simulink model "chbtask"  (R2024b)
settings: Solver=FixedStepDiscrete  StartTime=0.0  StopTime=0.2  FixedStep=5e-5  RelTol=1e-3
values from neighbouring files (symbols this model uses):
  CHB_MODE : value not decoded    [CHB_Data.sldd]
  INV120_CUURENTLOOP_KP = 2.0    [CHB_Data.sldd]
  INV120_CUURENTLOOP_KR = 5.0    [CHB_Data.sldd]
  INV120_VOLTAGELOOP_KI = 0.005    [CHB_Data.sldd]
  INV120_VOLTAGELOOP_KP = 0.5    [CHB_Data.sldd]
  INV240_VOLTAGELOOP_KI = 0.005    [CHB_Data.sldd]
  INV240_VOLTAGELOOP_KP = 0.5    [CHB_Data.sldd]
  PFC120_CUURENTLOOP_KP = 30.0    [CHB_Data.sldd]
  PFC120_CUURENTLOOP_KR = 8.0    [CHB_Data.sldd]
  PFC120_POWERLOOP_KI = 0.0001    [CHB_Data.sldd]
  PFC120_POWERLOOP_KP = 0.005    [CHB_Data.sldd]
  PFC240_CUURENTLOOP_KP = 5.0    [CHB_Data.sldd]
  PFC240_CUURENTLOOP_KR = 10.0    [CHB_Data.sldd]
  PFC240_POWERLOOP_KI = 0.0001    [CHB_Data.sldd]
  PFC240_POWERLOOP_KP = 0.005    [CHB_Data.sldd]
undefined symbols (not defined in the file or in its folder): Ii_rms, Io_rms, Io_rms_a, Io_rms_b, Vi_freq, Vi_rms, Vo_freq, Vo_freq_a, Vo_freq_b, Vo_rms, Vo_rms_a, Vo_rms_b
(part 3 of 3)

== stateflow chart chbtask/Algorithm_Ctrl/MainCtrl/inv120_func/inv120_en/Chart7 ==
  (default) -> (junction 3) : {
      | pi_out_value = single(1)*Pi_inv_out;
      | cnt = mod(cnt + 1, 200);
      | %PWM1 = sin_tab(mod(cnt + 0, 400) + 1);
      | out = pi_out_value*sin_wave(mod(cnt + 0, 200) + 1);
      | }
  data: sin_wave local single =[
0.000000000, 0.031410759, 0.062790520, 0.094108313, 0.125333234, 0.156434465, 0.187381315, 0.218143241, 0.248689887, 0.278991106, 0.309016994, 0.338737920, 0.368124553, 0.397147891, 0.425779292, 0.453990500, 0.481753674, 0.509041416, 0.535826795, 0.562083325, 0.587785252, 0.612907054, 0.637423990, 0.661311865, 0.684547106, 0.707106781, 0.728968627, 0.750111065, 0.770513243, 0.790155012, 0.809016994, 0.827080574, 0.844327926, 0.860742028, 0.876306680, 0.891006524, 0.904827052, 0.917754626, 0.929776486, 0.940880769, 0.951056516, 0.960293686, 0.968583162, 0.975916762, 0.982287251, 0.987688341, 0.992114701, 0.995561965, 0.998026728, 0.999506560, 1.000000000, 0.999506560, 0.998026728, 0.995561965, 0.992114701, 0.987688341, 0.982287251, 0.975916762, 0.968583162, 0.960293686, 0.951056516, 0.940880769, 0.929776486, 0.917754626, 0.904827052, 0.891006524, 0.876306680, 0.860742028, 0.844327926, 0.827080574, 0.809016994, 0.790155012, 0.770513243, 0.750111065, 0.728968627, 0.707106781, 0.684547106, 0.661311865, 0.637423990, 0.612907054, 0.587785252, 0.562083325, 0.535826795, 0.509041416, 0.481753674, 0.453990500, 0.425779292, 0.397147891, 0.368124553, 0.338737920, 0.309016994, 0.278991106, 0.248689887, 0.218143241, 0.187381315, 0.156434465, 0.125333234, 0.094108313, 0.062790520, 0.031410759, 0.000000000, -0.031410759, -0.062790520, -0.094108313, -0.125333234, -0.156434465, -0.187381315, -0.218143241, -0.248689887, -0.278991106, -0.309016994, -0.338737920, -0.368124553, -0.397147891, -0.425779292, -0.453990500, -0.481753674, -0.509041416, -0.535826795, -0.562083325, -0.587785252, -0.612907054, -0.637423990, -0.661311865, -0.684547106, -0.707106781, -0.728968627, -0.750111065, -0.770513243, -0.790155012, -0.809016994, -0.827080574, -0.844327926, -0.860742028, -0.876306680, -0.891006524, -0.904827052, -0.917754626, -0.929776486, -0.940880769, -0.951056516, -0.960293686, -0.968583162, -0.975916762, -0.982287251, -0.987688341, -0.992114701, -0.995561965, -0.998026728, -0.999506560, -1.000000000, -0.999506560, -0.998026728, -0.995561965, -0.992114701, -0.987688341, -0.982287251, -0.975916762, -0.968583162, -0.960293686, -0.951056516, -0.940880769, -0.929776486, -0.917754626, -0.904827052, -0.891006524, -0.876306680, -0.860742028, -0.844327926, -0.827080574, -0.809016994, -0.790155012, -0.770513243, -0.750111065, -0.728968627, -0.707106781, -0.684547106, -0.661311865, -0.637423990, -0.612907054, -0.587785252, -0.562083325, -0.535826795, -0.509041416, -0.481753674, -0.453990500, -0.425779292, -0.397147891, -0.368124553, -0.338737920, -0.309016994, -0.278991106, -0.248689887, -0.218143241, -0.187381315, -0.156434465, -0.125333234, -0.094108313, -0.062790520, -0.031410759
]; Pi_inv_out input single; cnt local single =0; out output single =0; pi_out_value local single =0

== stateflow chart chbtask/Task_Scheduler/Chart1 ==
  settings: executeAtInitialization=1
  (default) -> (junction 6)
  (junction 6) -> (junction 8) [order 1] : [cnt==0]
  (junction 6) -> (junction 11) [order 2] : {
      | out=0;
      | cnt=0;
      | }
  (junction 8) -> (junction 13) : {
      | out=1;
      | cnt=1;
      | }
  data: out output uint8 =0; cnt local uint8 =0
  events: event input FUNCTION_CALL_EVENT

== matlab function chbtask/Func/Rms/RMS ==
  data: Fs input single size=1; X_rms output single size=1; X_data input single size=1; limit_cnt input single size=[1 2]; pre_data input single size=[1 5]; X_freq output single size=1; out_data output single size=[1 5]
function [X_rms, X_freq, out_data] = RMS(Fs, X_data, limit_cnt, pre_data)
%%#codegen
sum_val = pre_data(1) + X_data * X_data; %均方根求和SUM
cnt = pre_data(2) + single(1); %cnt计数
prev = X_data;
out_data = [sum_val, cnt, prev, pre_data(4), pre_data(5)];

if (X_data > single(0)) && (pre_data(3) <= single(0)) && (cnt >= limit_cnt(1)) %过零点且采样点>最小限制
    temp = single(1) / cnt;
    X_freq = temp * Fs;
    X_rms = single(sqrt(double(temp * sum_val)));
    out_data(1) = single(0);
    out_data(2) = single(0);
    out_data(4) = X_rms;
    out_data(5) = X_freq;
elseif cnt > limit_cnt(2) %采样点>最大限制
    X_freq = single(0);
    X_rms = single(0);
    out_data(1) = single(0);
    out_data(2) = single(0);
    out_data(4) = single(0);
    out_data(5) = single(0);
else
    X_rms = pre_data(4);
    X_freq = pre_data(5);
end
end

== stateflow chart chbtask/Task_Scheduler/Chart ==
  state freq_divie
    %将系统频率分为20k、10k、5k、1k四个档次
    %%输出类型为事件触发
    cnt=cnt+1;
    %10k
    if (mod(cnt, 2)==0)
    freq_10k_flg1;
    elseif (mod(cnt, 2)==1)
    freq_10k_flg2;
    end
    %%5k
    if (mod(cnt, 4)==0)
    freq_05k_flg1;
    elseif(mod(cnt, 4)==1)
    freq_05k_flg2;
    elseif(mod(cnt, 4)==2)
    freq_5k_flg3;
    elseif(mod(cnt, 4)==3)
    freq_5k_flg4;
    elseif(mod(cnt, 4)==4)
    freq_5k_flg5;
    end
    %%1k
    if (mod(cnt, 20)==1)
    freq_01k_flg1;
    elseif(mod(cnt, 20)==2)
    freq_01k_flg2;
    elseif(mod(cnt, 20)==2)
    freq_01k_flg3;
    elseif(mod(cnt, 20)==2)
    freq_01k_flg4;
    elseif(mod(cnt, 20)==2)
    freq_01k_flg5;
    elseif(mod(cnt, 20)==0)
    cnt = 0;
    end
    freq_20k_flg;
  (default) -> freq_divie
  data: cnt local uint16 =0
  events: freq_01k_flg1 output FUNCTION_CALL_EVENT; freq_01k_flg2 output FUNCTION_CALL_EVENT; freq_01k_flg3 output FUNCTION_CALL_EVENT; freq_01k_flg4 output FUNCTION_CALL_EVENT; freq_01k_flg5 output FUNCTION_CALL_EVENT; freq_05k_flg1 output FUNCTION_CALL_EVENT; freq_05k_flg2 output FUNCTION_CALL_EVENT; freq_5k_flg3 output FUNCTION_CALL_EVENT; freq_5k_flg4 output FUNCTION_CALL_EVENT; freq_5k_flg5 output FUNCTION_CALL_EVENT; freq_10k_flg1 output FUNCTION_CALL_EVENT; freq_10k_flg2 output FUNCTION_CALL_EVENT; freq_20k_flg output FUNCTION_CALL_EVENT

== stateflow chart chbtask/SPWM_Table/SPWM_Chart ==
  state SPWM_gen
    entry:
    cnt = 0;
    during:
    cnt = mod(cnt + 1, 400);
    PWM1 = sin_tab(mod(cnt + 0, 400) + 1);
    PWM2 = 0.5 + 0.5*sin_tab(mod(cnt + 100, 400) + 1);
    PWM3 = 0.5 + 0.5*sin_tab(mod(cnt + 200, 400) + 1);
    PWM4 = 0.5 + 0.5*sin_tab(mod(cnt + 300, 400) + 1);
  data: PWM1 output single =0.5; PWM2 output single =0.99; PWM3 output single =0.5; PWM4 output single =0.01; cnt local int32; sin_tab local single =[0 0.0153931709655843 0.0307825438965657 0.0461643216954498 0.0615347091387271 0.076889913813288 0.092226147052144 0.107539624869224 0.122826568893018 0.138083207298831 0.153305775739426 0.168490518273821 0.18363368829401 0.198731549449382 0.213780376568612 0.228776456578787 0.243716089421558 0.258595588966065 0.273411283918445 0.288159518727658 0.302836654487448 0.317439069834186 0.331963161840386 0.346405346903672 0.360762061630984 0.375029763717788 0.389204932822085 0.403284071433007 0.417263705733771 0.431140386458797 0.444910689744756 0.458571217975362 0.472118600619681 0.485549495063759 0.498860587435364 0.51204859342163 0.525110259079417 0.538042361638169 0.550841710295088 0.563505147002413 0.576029547246624 0.588411820819366 0.600648912579917 0.612737803208991 0.624675509953716 0.63645908736358 0.648085628017179 0.659552263239578 0.670856163810115 0.681994540660468 0.692964645562816 0.703763771807925 0.714389254872983 0.724838473079037 0.73510884823785 0.74519784628803 0.755102977920273 0.764821799191563 0.774351912128177 0.783690965317349 0.792836654487448 0.801786723076523 0.810538962789071 0.819091214140905 0.827441366991975 0.83558736106701 0.843527186463865 0.851258884149428 0.858780546442986 0.86609031748692 0.8731863937046 0.880067024245403 0.886730511416699 0.893175211102736 0.899399533170302 0.905401941861061 0.911180956170486 0.91673515021327 0.922063153575141 0.927163651650994 0.93203538596925 0.936677154502364 0.941087811963404 0.945266270088642 0.949211497906058 0.952922521989723 0.956398426699972 0.95963835440933 0.962641505714115 0.965407139631678 0.967934573783235 0.970223184562226 0.972272407288188 0.974081736346076 0.975650725311018 0.976978987058465 0.978066193859706 0.978912077462731 0.979516429158417 0.979879099832027 0.98 0.979879099832027 0.979516429158417 0.978912077462731 0.978066193859706 0.976978987058465 0.975650725311018 0.974081736346076 0.972272407288188 0.970223184562226 0.967934573783235 0.965407139631678 0.962641505714115 0.95963835440933 0.956398426699972 0.952922521989723 0.949211497906058 0.945266270088642 0.941087811963404 0.936677154502364 0.932035385969251 0.927163651650994 0.922063153575141 0.91673515021327 0.911180956170486 0.905401941861061 0.899399533170302 0.893175211102736 0.886730511416699 0.880067024245403 0.8731863937046 0.86609031748692 0.858780546442986 0.851258884149427 0.843527186463865 0.83558736106701 0.827441366991975 0.819091214140905 0.81053896278907 0.801786723076523 0.792836654487448 0.783690965317349 0.774351912128176 0.764821799191563 0.755102977920273 0.74519784628803 0.73510884823785 0.724838473079037 0.714389254872983 0.703763771807925 0.692964645562817 0.681994540660468 0.670856163810115 0.659552263239578 0.648085628017179 0.63645908736358 0.624675509953716 0.612737803208991 0.600648912579917 0.588411820819366 0.576029547246624 0.563505147002413 0.550841710295088 0.538042361638169 0.525110259079417 0.51204859342163 0.498860587435364 0.485549495063759 0.472118600619681 0.458571217975362 0.444910689744756 0.431140386458797 0.417263705733771 0.403284071433007 0.389204932822085 0.375029763717788 0.360762061630985 0.346405346903672 0.331963161840385 0.317439069834186 0.302836654487449 0.288159518727658 0.273411283918445 0.258595588966066 0.243716089421558 0.228776456578787 0.213780376568612 0.198731549449382 0.18363368829401 0.168490518273821 0.153305775739426 0.138083207298831 0.122826568893018 0.107539624869225 0.0922261470521441 0.0768899138132882 0.0615347091387273 0.0461643216954501 0.0307825438965657 0.0153931709655843 1.20015386316441e-16 -0.0153931709655841 -0.0307825438965654 -0.0461643216954499 -0.0615347091387271 -0.0768899138132879 -0.0922261470521438 -0.107539624869224 -0.122826568893018 -0.138083207298831 -0.153305775739426 -0.168490518273821 -0.18363368829401 -0.198731549449382 -0.213780376568612 -0.228776456578787 -0.243716089421557 -0.258595588966065 -0.273411283918444 -0.288159518727658 -0.302836654487448 -0.317439069834187 -0.331963161840386 -0.346405346903672 -0.360762061630984 -0.375029763717788 -0.389204932822085 -0.403284071433006 -0.417263705733771 -0.431140386458796 -0.444910689744756 -0.458571217975362 -0.472118600619681 -0.485549495063759 -0.498860587435364 -0.51204859342163 -0.525110259079416 -0.538042361638169 -0.550841710295088 -0.563505147002412 -0.576029547246623 -0.588411820819366 -0.600648912579917 -0.612737803208991 -0.624675509953716 -0.63645908736358 -0.648085628017179 -0.659552263239578 -0.670856163810115 -0.681994540660468 -0.692964645562816 -0.703763771807925 -0.714389254872983 -0.724838473079037 -0.73510884823785 -0.745197846288031 -0.755102977920274 -0.764821799191563 -0.774351912128177 -0.783690965317349 -0.792836654487448 -0.801786723076523 -0.81053896278907 -0.819091214140905 -0.827441366991975 -0.835587361067011 -0.843527186463865 -0.851258884149428 -0.858780546442986 -0.866090317486919 -0.8731863937046 -0.880067024245403 -0.886730511416699 -0.893175211102736 -0.899399533170302 -0.905401941861061 -0.911180956170486 -0.91673515021327 -0.922063153575141 -0.927163651650994 -0.93203538596925 -0.936677154502363 -0.941087811963404 -0.945266270088642 -0.949211497906059 -0.952922521989723 -0.956398426699972 -0.95963835440933 -0.962641505714115 -0.965407139631678 -0.967934573783235 -0.970223184562226 -0.972272407288188 -0.974081736346076 -0.975650725311018 -0.976978987058465 -0.978066193859706 -0.978912077462731 -0.979516429158417 -0.979879099832027 -0.98 -0.979879099832027 -0.979516429158417 -0.978912077462731 -0.978066193859706 -0.976978987058465 -0.975650725311018 -0.974081736346076 -0.972272407288188 -0.970223184562226 -0.967934573783235 -0.965407139631678 -0.962641505714115 -0.959638354409331 -0.956398426699973 -0.952922521989723 -0.949211497906058 -0.945266270088642 -0.941087811963404 -0.936677154502364 -0.932035385969251 -0.927163651650994 -0.922063153575141 -0.91673515021327 -0.911180956170487 -0.905401941861061 -0.899399533170302 -0.893175211102736 -0.886730511416699 -0.880067024245403 -0.873186393704601 -0.86609031748692 -0.858780546442986 -0.851258884149428 -0.843527186463864 -0.835587361067011 -0.827441366991975 -0.819091214140905 -0.810538962789071 -0.801786723076523 -0.792836654487449 -0.783690965317349 -0.774351912128177 -0.764821799191563 -0.755102977920274 -0.74519784628803 -0.735108848237851 -0.724838473079037 -0.714389254872984 -0.703763771807925 -0.692964645562817 -0.681994540660468 -0.670856163810115 -0.659552263239578 -0.648085628017179 -0.63645908736358 -0.624675509953716 -0.612737803208992 -0.600648912579917 -0.588411820819367 -0.576029547246624 -0.563505147002413 -0.550841710295088 -0.538042361638169 -0.525110259079417 -0.51204859342163 -0.498860587435365 -0.485549495063759 -0.472118600619682 -0.458571217975362 -0.444910689744756 -0.431140386458797 -0.417263705733772 -0.403284071433007 -0.389204932822085 -0.375029763717789 -0.360762061630984 -0.346405346903673 -0.331963161840386 -0.317439069834187 -0.302836654487449 -0.288159518727658 -0.273411283918445 -0.258595588966066 -0.243716089421558 -0.228776456578787 -0.213780376568612 -0.198731549449382 -0.18363368829401 -0.168490518273821 -0.153305775739426 -0.138083207298831 -0.122826568893019 -0.107539624869225 -0.0922261470521446 -0.0768899138132887 -0.061534709138727 -0.0461643216954498 -0.0307825438965658 -0.0153931709655844]
